simulink model "test"  (Simulink 7.0)
settings: Solver=FixedStepDiscrete  StartTime=0.0  StopTime=10  FixedStep=.1  RelTol=1e-3
libraries: dsPICdrivers x5
settings Model: Creator=sicard  LastModifiedBy=atoubi
settings OptimizationCC: InlineParams=on  InlineInvariantSignals=on  EnforceIntegerDowncast=off  StateBitsets=on  DataBitsets=on  UseTempVars=on  ZeroExternalMemoryAtStartup=off  ZeroInternalMemoryAtStartup=off  InitFltsAndDblsToZero=off  OptimizeModelRefInitCode=on  LifeSpan=1
settings DebuggingCC: InheritedTsInSrcMsg=none
settings HardwareCC: ProdBitPerInt=16  ProdEndianess=LittleEndian  ProdWordSize=16  ProdHWDeviceType=16-bit Generic  TargetHWDeviceType=32-bit Generic
settings RTWCC: SystemTargetFile=dspic.tlc  TemplateMakefile=dspic_pic30_gcc.tmf  PostCodeGenCommand=dsPIC_Compile()  Description=Embedded Target for Microchip dsPIC (real-time)  ProcessScript=dspic_make_rtw_hook
settings CodeAppCC: IgnoreCustomStorageClasses=off
settings STFCustomTargetCC: GenFloatMathFcnCalls=ANSI_C  ModelReferenceCompliant=off  IncludeMdlTerminateFcn=off  CombineOutputUpdateFcns=on  SuppressErrorStatus=on  ERTCustomFileBanners=on  SupportContinuousTime=off  SupportNonInlinedSFcns=off  SystemTargetFile=dspic.tlc
settings ERTTargetCC: GenFloatMathFcnCalls=ANSI_C  ModelReferenceCompliant=off  CompOptLevelCompliant=off  IncludeMdlTerminateFcn=off  SuppressErrorStatus=on  ModelStepFunctionPrototypeControlCompliant=off  ExtModeMexFile=noextcomm  InlinedParameterPlacement=NonHierarchical  ERTSrcFileBannerTemplate=dsPIC_code_template.cgt  ERTHdrFileBannerTemplate=dsPIC_code_template.cgt  ERTDataSrcFileTemplate=dsPIC_code_template.cgt  ERTDataHdrFileTemplate=dsPIC_code_template.cgt  ERTCustomFileTemplate=dsPIC_main.tlc
settings CustomProperty: DataType=string  Value=C:\PROGRA~1\MATLAB1\R2007b\bin\win32\gmake

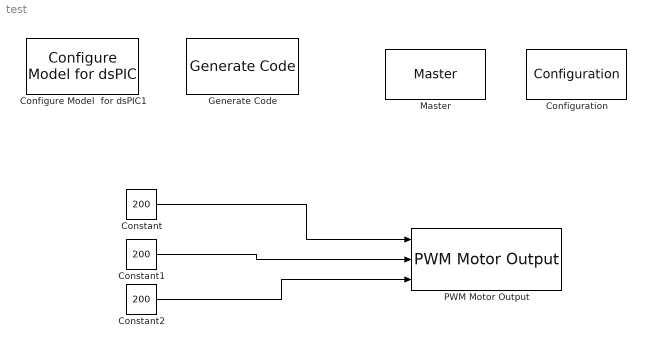
== system test ==
  Configuration : dsPICdrivers/Configuration  SystemSampleTime=-1  double64=off
  Configure Model  for dsPIC1 : dsPICdrivers/Simulink Configuration/Configure Model  for dsPIC
  Constant : Constant  Value=200  OutDataTypeMode=uint16  OutDataType=sfix(16)  OutScaling=2^0
  Constant1 : Constant  Value=200  OutDataTypeMode=uint16  OutDataType=sfix(16)  OutScaling=2^0
  Constant2 : Constant  Value=200  OutDataTypeMode=uint16  OutDataType=sfix(16)  OutScaling=2^0
  Generate Code : dsPICdrivers/Simulink Configuration/Generate Code
  Master : dsPICdrivers/Master  Tag=dsPIC_MASTER  Priority=1  TimeStepType=Timer1  picType=33fj32MC302  fcy=40000000  Quartz_33f=20e6  PLLActive_33f=on  fcyDesired_33f=40e6  tmr1="[64  62499  0]"  tmr1Info="Time Step : 0.1  ;   Error : 0%  PR1=62499"  tmr2345="[0  0  0  0]"  tmr2345cfg=[-1 -1 -1 -1]  IOautoConf=on  typePort="[ 0  0  0  0  0  0  0  0  0  0  0  0  0  0  0  0  0  0  0  0  0  0  0  0  0  0  0  0  0  0  0  0  0  0  0  0  0  0  0  0  0  0  0  0  0  0  0  0  0  0  0  0  0  0  0  0  0  0  0  0  0  0  0  0  0  0  0  0  0  0  0  0  0  0  0  0  0  0  0  0  0  0  0  0  0  0  0  0  0  0  0  0  0  0  0  0  0  0  0  0  0  0  0  0  0  0  0  0  0  0  0  0 ]"  TRIS="[ 65535  65535  65535  65535  65535  65535  65535 ]"  ADPCFG=0  MasterBusyPort=None  MasterOverloadPort=None  FOSC=Quartz (XT - HS)  ClockSwitchMonitor=Both disabled  TempProtection_33f=TEMP_ON  FPBOR=<empty>  PWRT=disable  MCLR=<empty>  ICD=ICS_NONE  JTAGEN=JTAGEN_OFF  PowerSave=off  OverrideFcy=off  NewFcy=1e6  PR2345="[65535  65535  65535  65535]"
  PWM Motor Output : dsPICdrivers/Peripheral I//O/PWM Motor Output  Tag=dsPIC_PWM_Motor  Priority=5  PWMref=1  PWM12=2  InputEnableChk=off  InputPeriodeChk=off  Channel=[1 2 3]  TPeriode=1e-4  PrescalerValue=1  PeriodeInteger=2000  MaxName='PWM'  Centered=on  HChannelON=off  Info="Nbr Bits : 11.9658  ||  PWM = 4000  ||  Prescaler = 1"  Delay=0  IntPriority=5  nbrPwmChannelPIC=3  Status=OK  DeadTimePrescaleA=0  DeadTimePrescaleB=0  DeadTimeInfo="Dead Time A = 0  ||  Dead Time B = 0"  DTPWM1a=Prescaler A  DTPWM1i=Prescaler A  DTPWM2a=Prescaler A  DTPWM2i=Prescaler A  DTPWM3a=Prescaler A  DTPWM3i=Prescaler A  DTPWM4a=Prescaler A  DTPWM4i=Prescaler A  DTCON1=0  DTCON2=0
  wires:
  Constant/1 -> PWM Motor Output/1
  Constant1/1 -> PWM Motor Output/2
  Constant2/1 -> PWM Motor Output/3
